simulink model "WarehouseFleetSim"  (R2024b)
settings: Solver=ode4  StartTime=0.0  StopTime=inf  FixedStep=0.02  RelTol=1e-3
StopFcn:
  | try, fleetVisionStep('close'); catch, end; try, phase3('stopped'); catch, end
model workspace (MAT data in the model file):
  HomePose1 = [-20 7.3 0]
  HomePose2 = [-20 3.6 0]
  HomePose3 = [-20 11 0]
  HomePose4 = [-24.5 3.6 0]
  HomePose5 = [-24.5 7.3 0]
  HomePose6 = [-24.5 11 0]
  Zero = 0
  gen3 : robotics.RigidBodyTree (value not decoded)
  qStow = [0; 0; 0.261799387799; 3.14159265359; -2.26892802759; 0; 0.959931088597; 1.57079632679]
undefined symbols (not defined in the file or in its folder): Actor, setupFleetScene, Sim3dSensor, World
libraries: sim3dlib x128, sim3dcameralib x7, robotmobilelib x6, robotsim3dlib x6
(part 2 of 4)

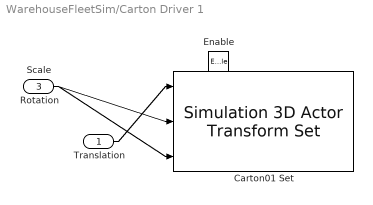
== system WarehouseFleetSim/Carton Driver 1 ==
  Translation : Inport
  Rotation : Inport  Port=2
  Scale : Inport  Port=3
  Enable : EnablePort
  Carton01 Set : sim3dlib/Simulation 3D Actor Transform Set  Priority=1  ActorTag=Carton01  NumberOfParts=1  CustNumOfParts=3  Translation=[0 0 0]  Rotation=[0 0 0]  Scale=[1 1 1]  Ts=-1  aMode=aMode
  wires:
  Translation/1 -> Carton01 Set/1
  Rotation/1 -> Carton01 Set/2
  Scale/1 -> Carton01 Set/3

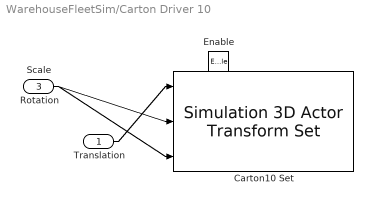
== system WarehouseFleetSim/Carton Driver 10 ==
  Translation : Inport
  Rotation : Inport  Port=2
  Scale : Inport  Port=3
  Enable : EnablePort
  Carton10 Set : sim3dlib/Simulation 3D Actor Transform Set  Priority=1  ActorTag=Carton10  NumberOfParts=1  CustNumOfParts=3  Translation=[0 0 0]  Rotation=[0 0 0]  Scale=[1 1 1]  Ts=-1  aMode=aMode
  wires:
  Translation/1 -> Carton10 Set/1
  Rotation/1 -> Carton10 Set/2
  Scale/1 -> Carton10 Set/3

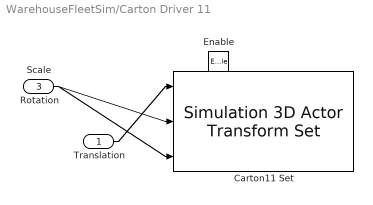
== system WarehouseFleetSim/Carton Driver 11 ==
  Translation : Inport
  Rotation : Inport  Port=2
  Scale : Inport  Port=3
  Enable : EnablePort
  Carton11 Set : sim3dlib/Simulation 3D Actor Transform Set  Priority=1  ActorTag=Carton11  NumberOfParts=1  CustNumOfParts=3  Translation=[0 0 0]  Rotation=[0 0 0]  Scale=[1 1 1]  Ts=-1  aMode=aMode
  wires:
  Translation/1 -> Carton11 Set/1
  Rotation/1 -> Carton11 Set/2
  Scale/1 -> Carton11 Set/3

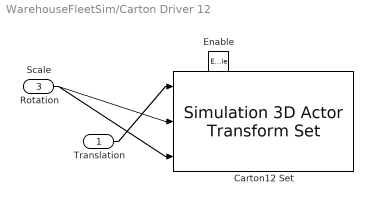
== system WarehouseFleetSim/Carton Driver 12 ==
  Translation : Inport
  Rotation : Inport  Port=2
  Scale : Inport  Port=3
  Enable : EnablePort
  Carton12 Set : sim3dlib/Simulation 3D Actor Transform Set  Priority=1  ActorTag=Carton12  NumberOfParts=1  CustNumOfParts=3  Translation=[0 0 0]  Rotation=[0 0 0]  Scale=[1 1 1]  Ts=-1  aMode=aMode
  wires:
  Translation/1 -> Carton12 Set/1
  Rotation/1 -> Carton12 Set/2
  Scale/1 -> Carton12 Set/3

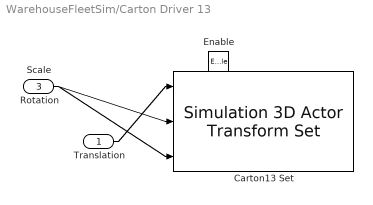
== system WarehouseFleetSim/Carton Driver 13 ==
  Translation : Inport
  Rotation : Inport  Port=2
  Scale : Inport  Port=3
  Enable : EnablePort
  Carton13 Set : sim3dlib/Simulation 3D Actor Transform Set  Priority=1  ActorTag=Carton13  NumberOfParts=1  CustNumOfParts=3  Translation=[0 0 0]  Rotation=[0 0 0]  Scale=[1 1 1]  Ts=-1  aMode=aMode
  wires:
  Translation/1 -> Carton13 Set/1
  Rotation/1 -> Carton13 Set/2
  Scale/1 -> Carton13 Set/3

== system WarehouseFleetSim/Carton Driver 14 ==
  Translation : Inport
  Rotation : Inport  Port=2
  Scale : Inport  Port=3
  Enable : EnablePort
  Carton14 Set : sim3dlib/Simulation 3D Actor Transform Set  Priority=1  ActorTag=Carton14  NumberOfParts=1  CustNumOfParts=3  Translation=[0 0 0]  Rotation=[0 0 0]  Scale=[1 1 1]  Ts=-1  aMode=aMode
  wires:
  Translation/1 -> Carton14 Set/1
  Rotation/1 -> Carton14 Set/2
  Scale/1 -> Carton14 Set/3

== system WarehouseFleetSim/Carton Driver 15 ==
  Translation : Inport
  Rotation : Inport  Port=2
  Scale : Inport  Port=3
  Enable : EnablePort
  Carton15 Set : sim3dlib/Simulation 3D Actor Transform Set  Priority=1  ActorTag=Carton15  NumberOfParts=1  CustNumOfParts=3  Translation=[0 0 0]  Rotation=[0 0 0]  Scale=[1 1 1]  Ts=-1  aMode=aMode
  wires:
  Translation/1 -> Carton15 Set/1
  Rotation/1 -> Carton15 Set/2
  Scale/1 -> Carton15 Set/3

== system WarehouseFleetSim/Carton Driver 16 ==
  Translation : Inport
  Rotation : Inport  Port=2
  Scale : Inport  Port=3
  Enable : EnablePort
  Carton16 Set : sim3dlib/Simulation 3D Actor Transform Set  Priority=1  ActorTag=Carton16  NumberOfParts=1  CustNumOfParts=3  Translation=[0 0 0]  Rotation=[0 0 0]  Scale=[1 1 1]  Ts=-1  aMode=aMode
  wires:
  Translation/1 -> Carton16 Set/1
  Rotation/1 -> Carton16 Set/2
  Scale/1 -> Carton16 Set/3

== system WarehouseFleetSim/Carton Driver 17 ==
  Translation : Inport
  Rotation : Inport  Port=2
  Scale : Inport  Port=3
  Enable : EnablePort
  Carton17 Set : sim3dlib/Simulation 3D Actor Transform Set  Priority=1  ActorTag=Carton17  NumberOfParts=1  CustNumOfParts=3  Translation=[0 0 0]  Rotation=[0 0 0]  Scale=[1 1 1]  Ts=-1  aMode=aMode
  wires:
  Translation/1 -> Carton17 Set/1
  Rotation/1 -> Carton17 Set/2
  Scale/1 -> Carton17 Set/3

== system WarehouseFleetSim/Carton Driver 18 ==
  Translation : Inport
  Rotation : Inport  Port=2
  Scale : Inport  Port=3
  Enable : EnablePort
  Carton18 Set : sim3dlib/Simulation 3D Actor Transform Set  Priority=1  ActorTag=Carton18  NumberOfParts=1  CustNumOfParts=3  Translation=[0 0 0]  Rotation=[0 0 0]  Scale=[1 1 1]  Ts=-1  aMode=aMode
  wires:
  Translation/1 -> Carton18 Set/1
  Rotation/1 -> Carton18 Set/2
  Scale/1 -> Carton18 Set/3

== system WarehouseFleetSim/Carton Driver 19 ==
  Translation : Inport
  Rotation : Inport  Port=2
  Scale : Inport  Port=3
  Enable : EnablePort
  Carton19 Set : sim3dlib/Simulation 3D Actor Transform Set  Priority=1  ActorTag=Carton19  NumberOfParts=1  CustNumOfParts=3  Translation=[0 0 0]  Rotation=[0 0 0]  Scale=[1 1 1]  Ts=-1  aMode=aMode
  wires:
  Translation/1 -> Carton19 Set/1
  Rotation/1 -> Carton19 Set/2
  Scale/1 -> Carton19 Set/3

== system WarehouseFleetSim/Carton Driver 2 ==
  Translation : Inport
  Rotation : Inport  Port=2
  Scale : Inport  Port=3
  Enable : EnablePort
  Carton02 Set : sim3dlib/Simulation 3D Actor Transform Set  Priority=1  ActorTag=Carton02  NumberOfParts=1  CustNumOfParts=3  Translation=[0 0 0]  Rotation=[0 0 0]  Scale=[1 1 1]  Ts=-1  aMode=aMode
  wires:
  Translation/1 -> Carton02 Set/1
  Rotation/1 -> Carton02 Set/2
  Scale/1 -> Carton02 Set/3

== system WarehouseFleetSim/Carton Driver 20 ==
  Translation : Inport
  Rotation : Inport  Port=2
  Scale : Inport  Port=3
  Enable : EnablePort
  Carton20 Set : sim3dlib/Simulation 3D Actor Transform Set  Priority=1  ActorTag=Carton20  NumberOfParts=1  CustNumOfParts=3  Translation=[0 0 0]  Rotation=[0 0 0]  Scale=[1 1 1]  Ts=-1  aMode=aMode
  wires:
  Translation/1 -> Carton20 Set/1
  Rotation/1 -> Carton20 Set/2
  Scale/1 -> Carton20 Set/3

== system WarehouseFleetSim/Carton Driver 21 ==
  Translation : Inport
  Rotation : Inport  Port=2
  Scale : Inport  Port=3
  Enable : EnablePort
  Carton21 Set : sim3dlib/Simulation 3D Actor Transform Set  Priority=1  ActorTag=Carton21  NumberOfParts=1  CustNumOfParts=3  Translation=[0 0 0]  Rotation=[0 0 0]  Scale=[1 1 1]  Ts=-1  aMode=aMode
  wires:
  Translation/1 -> Carton21 Set/1
  Rotation/1 -> Carton21 Set/2
  Scale/1 -> Carton21 Set/3

== system WarehouseFleetSim/Carton Driver 22 ==
  Translation : Inport
  Rotation : Inport  Port=2
  Scale : Inport  Port=3
  Enable : EnablePort
  Carton22 Set : sim3dlib/Simulation 3D Actor Transform Set  Priority=1  ActorTag=Carton22  NumberOfParts=1  CustNumOfParts=3  Translation=[0 0 0]  Rotation=[0 0 0]  Scale=[1 1 1]  Ts=-1  aMode=aMode
  wires:
  Translation/1 -> Carton22 Set/1
  Rotation/1 -> Carton22 Set/2
  Scale/1 -> Carton22 Set/3

== system WarehouseFleetSim/Carton Driver 23 ==
  Translation : Inport
  Rotation : Inport  Port=2
  Scale : Inport  Port=3
  Enable : EnablePort
  Carton23 Set : sim3dlib/Simulation 3D Actor Transform Set  Priority=1  ActorTag=Carton23  NumberOfParts=1  CustNumOfParts=3  Translation=[0 0 0]  Rotation=[0 0 0]  Scale=[1 1 1]  Ts=-1  aMode=aMode
  wires:
  Translation/1 -> Carton23 Set/1
  Rotation/1 -> Carton23 Set/2
  Scale/1 -> Carton23 Set/3

== system WarehouseFleetSim/Carton Driver 24 ==
  Translation : Inport
  Rotation : Inport  Port=2
  Scale : Inport  Port=3
  Enable : EnablePort
  Carton24 Set : sim3dlib/Simulation 3D Actor Transform Set  Priority=1  ActorTag=Carton24  NumberOfParts=1  CustNumOfParts=3  Translation=[0 0 0]  Rotation=[0 0 0]  Scale=[1 1 1]  Ts=-1  aMode=aMode
  wires:
  Translation/1 -> Carton24 Set/1
  Rotation/1 -> Carton24 Set/2
  Scale/1 -> Carton24 Set/3

== system WarehouseFleetSim/Carton Driver 25 ==
  Translation : Inport
  Rotation : Inport  Port=2
  Scale : Inport  Port=3
  Enable : EnablePort
  Carton25 Set : sim3dlib/Simulation 3D Actor Transform Set  Priority=1  ActorTag=Carton25  NumberOfParts=1  CustNumOfParts=3  Translation=[0 0 0]  Rotation=[0 0 0]  Scale=[1 1 1]  Ts=-1  aMode=aMode
  wires:
  Translation/1 -> Carton25 Set/1
  Rotation/1 -> Carton25 Set/2
  Scale/1 -> Carton25 Set/3

== system WarehouseFleetSim/Carton Driver 26 ==
  Translation : Inport
  Rotation : Inport  Port=2
  Scale : Inport  Port=3
  Enable : EnablePort
  Carton26 Set : sim3dlib/Simulation 3D Actor Transform Set  Priority=1  ActorTag=Carton26  NumberOfParts=1  CustNumOfParts=3  Translation=[0 0 0]  Rotation=[0 0 0]  Scale=[1 1 1]  Ts=-1  aMode=aMode
  wires:
  Translation/1 -> Carton26 Set/1
  Rotation/1 -> Carton26 Set/2
  Scale/1 -> Carton26 Set/3

== system WarehouseFleetSim/Carton Driver 27 ==
  Translation : Inport
  Rotation : Inport  Port=2
  Scale : Inport  Port=3
  Enable : EnablePort
  Carton27 Set : sim3dlib/Simulation 3D Actor Transform Set  Priority=1  ActorTag=Carton27  NumberOfParts=1  CustNumOfParts=3  Translation=[0 0 0]  Rotation=[0 0 0]  Scale=[1 1 1]  Ts=-1  aMode=aMode
  wires:
  Translation/1 -> Carton27 Set/1
  Rotation/1 -> Carton27 Set/2
  Scale/1 -> Carton27 Set/3

== system WarehouseFleetSim/Carton Driver 28 ==
  Translation : Inport
  Rotation : Inport  Port=2
  Scale : Inport  Port=3
  Enable : EnablePort
  Carton28 Set : sim3dlib/Simulation 3D Actor Transform Set  Priority=1  ActorTag=Carton28  NumberOfParts=1  CustNumOfParts=3  Translation=[0 0 0]  Rotation=[0 0 0]  Scale=[1 1 1]  Ts=-1  aMode=aMode
  wires:
  Translation/1 -> Carton28 Set/1
  Rotation/1 -> Carton28 Set/2
  Scale/1 -> Carton28 Set/3

== system WarehouseFleetSim/Carton Driver 29 ==
  Translation : Inport
  Rotation : Inport  Port=2
  Scale : Inport  Port=3
  Enable : EnablePort
  Carton29 Set : sim3dlib/Simulation 3D Actor Transform Set  Priority=1  ActorTag=Carton29  NumberOfParts=1  CustNumOfParts=3  Translation=[0 0 0]  Rotation=[0 0 0]  Scale=[1 1 1]  Ts=-1  aMode=aMode
  wires:
  Translation/1 -> Carton29 Set/1
  Rotation/1 -> Carton29 Set/2
  Scale/1 -> Carton29 Set/3

== system WarehouseFleetSim/Carton Driver 3 ==
  Translation : Inport
  Rotation : Inport  Port=2
  Scale : Inport  Port=3
  Enable : EnablePort
  Carton03 Set : sim3dlib/Simulation 3D Actor Transform Set  Priority=1  ActorTag=Carton03  NumberOfParts=1  CustNumOfParts=3  Translation=[0 0 0]  Rotation=[0 0 0]  Scale=[1 1 1]  Ts=-1  aMode=aMode
  wires:
  Translation/1 -> Carton03 Set/1
  Rotation/1 -> Carton03 Set/2
  Scale/1 -> Carton03 Set/3

== system WarehouseFleetSim/Carton Driver 30 ==
  Translation : Inport
  Rotation : Inport  Port=2
  Scale : Inport  Port=3
  Enable : EnablePort
  Carton30 Set : sim3dlib/Simulation 3D Actor Transform Set  Priority=1  ActorTag=Carton30  NumberOfParts=1  CustNumOfParts=3  Translation=[0 0 0]  Rotation=[0 0 0]  Scale=[1 1 1]  Ts=-1  aMode=aMode
  wires:
  Translation/1 -> Carton30 Set/1
  Rotation/1 -> Carton30 Set/2
  Scale/1 -> Carton30 Set/3

== system WarehouseFleetSim/Carton Driver 31 ==
  Translation : Inport
  Rotation : Inport  Port=2
  Scale : Inport  Port=3
  Enable : EnablePort
  Carton31 Set : sim3dlib/Simulation 3D Actor Transform Set  Priority=1  ActorTag=Carton31  NumberOfParts=1  CustNumOfParts=3  Translation=[0 0 0]  Rotation=[0 0 0]  Scale=[1 1 1]  Ts=-1  aMode=aMode
  wires:
  Translation/1 -> Carton31 Set/1
  Rotation/1 -> Carton31 Set/2
  Scale/1 -> Carton31 Set/3

== system WarehouseFleetSim/Carton Driver 32 ==
  Translation : Inport
  Rotation : Inport  Port=2
  Scale : Inport  Port=3
  Enable : EnablePort
  Carton32 Set : sim3dlib/Simulation 3D Actor Transform Set  Priority=1  ActorTag=Carton32  NumberOfParts=1  CustNumOfParts=3  Translation=[0 0 0]  Rotation=[0 0 0]  Scale=[1 1 1]  Ts=-1  aMode=aMode
  wires:
  Translation/1 -> Carton32 Set/1
  Rotation/1 -> Carton32 Set/2
  Scale/1 -> Carton32 Set/3

== system WarehouseFleetSim/Carton Driver 33 ==
  Translation : Inport
  Rotation : Inport  Port=2
  Scale : Inport  Port=3
  Enable : EnablePort
  Carton33 Set : sim3dlib/Simulation 3D Actor Transform Set  Priority=1  ActorTag=Carton33  NumberOfParts=1  CustNumOfParts=3  Translation=[0 0 0]  Rotation=[0 0 0]  Scale=[1 1 1]  Ts=-1  aMode=aMode
  wires:
  Translation/1 -> Carton33 Set/1
  Rotation/1 -> Carton33 Set/2
  Scale/1 -> Carton33 Set/3

== system WarehouseFleetSim/Carton Driver 34 ==
  Translation : Inport
  Rotation : Inport  Port=2
  Scale : Inport  Port=3
  Enable : EnablePort
  Carton34 Set : sim3dlib/Simulation 3D Actor Transform Set  Priority=1  ActorTag=Carton34  NumberOfParts=1  CustNumOfParts=3  Translation=[0 0 0]  Rotation=[0 0 0]  Scale=[1 1 1]  Ts=-1  aMode=aMode
  wires:
  Translation/1 -> Carton34 Set/1
  Rotation/1 -> Carton34 Set/2
  Scale/1 -> Carton34 Set/3

== system WarehouseFleetSim/Carton Driver 35 ==
  Translation : Inport
  Rotation : Inport  Port=2
  Scale : Inport  Port=3
  Enable : EnablePort
  Carton35 Set : sim3dlib/Simulation 3D Actor Transform Set  Priority=1  ActorTag=Carton35  NumberOfParts=1  CustNumOfParts=3  Translation=[0 0 0]  Rotation=[0 0 0]  Scale=[1 1 1]  Ts=-1  aMode=aMode
  wires:
  Translation/1 -> Carton35 Set/1
  Rotation/1 -> Carton35 Set/2
  Scale/1 -> Carton35 Set/3

== system WarehouseFleetSim/Carton Driver 36 ==
  Translation : Inport
  Rotation : Inport  Port=2
  Scale : Inport  Port=3
  Enable : EnablePort
  Carton36 Set : sim3dlib/Simulation 3D Actor Transform Set  Priority=1  ActorTag=Carton36  NumberOfParts=1  CustNumOfParts=3  Translation=[0 0 0]  Rotation=[0 0 0]  Scale=[1 1 1]  Ts=-1  aMode=aMode
  wires:
  Translation/1 -> Carton36 Set/1
  Rotation/1 -> Carton36 Set/2
  Scale/1 -> Carton36 Set/3

== system WarehouseFleetSim/Carton Driver 37 ==
  Translation : Inport
  Rotation : Inport  Port=2
  Scale : Inport  Port=3
  Enable : EnablePort
  Carton37 Set : sim3dlib/Simulation 3D Actor Transform Set  Priority=1  ActorTag=Carton37  NumberOfParts=1  CustNumOfParts=3  Translation=[0 0 0]  Rotation=[0 0 0]  Scale=[1 1 1]  Ts=-1  aMode=aMode
  wires:
  Translation/1 -> Carton37 Set/1
  Rotation/1 -> Carton37 Set/2
  Scale/1 -> Carton37 Set/3

== system WarehouseFleetSim/Carton Driver 38 ==
  Translation : Inport
  Rotation : Inport  Port=2
  Scale : Inport  Port=3
  Enable : EnablePort
  Carton38 Set : sim3dlib/Simulation 3D Actor Transform Set  Priority=1  ActorTag=Carton38  NumberOfParts=1  CustNumOfParts=3  Translation=[0 0 0]  Rotation=[0 0 0]  Scale=[1 1 1]  Ts=-1  aMode=aMode
  wires:
  Translation/1 -> Carton38 Set/1
  Rotation/1 -> Carton38 Set/2
  Scale/1 -> Carton38 Set/3

== system WarehouseFleetSim/Carton Driver 39 ==
  Translation : Inport
  Rotation : Inport  Port=2
  Scale : Inport  Port=3
  Enable : EnablePort
  Carton39 Set : sim3dlib/Simulation 3D Actor Transform Set  Priority=1  ActorTag=Carton39  NumberOfParts=1  CustNumOfParts=3  Translation=[0 0 0]  Rotation=[0 0 0]  Scale=[1 1 1]  Ts=-1  aMode=aMode
  wires:
  Translation/1 -> Carton39 Set/1
  Rotation/1 -> Carton39 Set/2
  Scale/1 -> Carton39 Set/3

== system WarehouseFleetSim/Carton Driver 4 ==
  Translation : Inport
  Rotation : Inport  Port=2
  Scale : Inport  Port=3
  Enable : EnablePort
  Carton04 Set : sim3dlib/Simulation 3D Actor Transform Set  Priority=1  ActorTag=Carton04  NumberOfParts=1  CustNumOfParts=3  Translation=[0 0 0]  Rotation=[0 0 0]  Scale=[1 1 1]  Ts=-1  aMode=aMode
  wires:
  Translation/1 -> Carton04 Set/1
  Rotation/1 -> Carton04 Set/2
  Scale/1 -> Carton04 Set/3

== system WarehouseFleetSim/Carton Driver 40 ==
  Translation : Inport
  Rotation : Inport  Port=2
  Scale : Inport  Port=3
  Enable : EnablePort
  Carton40 Set : sim3dlib/Simulation 3D Actor Transform Set  Priority=1  ActorTag=Carton40  NumberOfParts=1  CustNumOfParts=3  Translation=[0 0 0]  Rotation=[0 0 0]  Scale=[1 1 1]  Ts=-1  aMode=aMode
  wires:
  Translation/1 -> Carton40 Set/1
  Rotation/1 -> Carton40 Set/2
  Scale/1 -> Carton40 Set/3

== system WarehouseFleetSim/Carton Driver 41 ==
  Translation : Inport
  Rotation : Inport  Port=2
  Scale : Inport  Port=3
  Enable : EnablePort
  Carton41 Set : sim3dlib/Simulation 3D Actor Transform Set  Priority=1  ActorTag=Carton41  NumberOfParts=1  CustNumOfParts=3  Translation=[0 0 0]  Rotation=[0 0 0]  Scale=[1 1 1]  Ts=-1  aMode=aMode
  wires:
  Translation/1 -> Carton41 Set/1
  Rotation/1 -> Carton41 Set/2
  Scale/1 -> Carton41 Set/3

== system WarehouseFleetSim/Carton Driver 42 ==
  Translation : Inport
  Rotation : Inport  Port=2
  Scale : Inport  Port=3
  Enable : EnablePort
  Carton42 Set : sim3dlib/Simulation 3D Actor Transform Set  Priority=1  ActorTag=Carton42  NumberOfParts=1  CustNumOfParts=3  Translation=[0 0 0]  Rotation=[0 0 0]  Scale=[1 1 1]  Ts=-1  aMode=aMode
  wires:
  Translation/1 -> Carton42 Set/1
  Rotation/1 -> Carton42 Set/2
  Scale/1 -> Carton42 Set/3

== system WarehouseFleetSim/Carton Driver 43 ==
  Translation : Inport
  Rotation : Inport  Port=2
  Scale : Inport  Port=3
  Enable : EnablePort
  Carton43 Set : sim3dlib/Simulation 3D Actor Transform Set  Priority=1  ActorTag=Carton43  NumberOfParts=1  CustNumOfParts=3  Translation=[0 0 0]  Rotation=[0 0 0]  Scale=[1 1 1]  Ts=-1  aMode=aMode
  wires:
  Translation/1 -> Carton43 Set/1
  Rotation/1 -> Carton43 Set/2
  Scale/1 -> Carton43 Set/3

== system WarehouseFleetSim/Carton Driver 44 ==
  Translation : Inport
  Rotation : Inport  Port=2
  Scale : Inport  Port=3
  Enable : EnablePort
  Carton44 Set : sim3dlib/Simulation 3D Actor Transform Set  Priority=1  ActorTag=Carton44  NumberOfParts=1  CustNumOfParts=3  Translation=[0 0 0]  Rotation=[0 0 0]  Scale=[1 1 1]  Ts=-1  aMode=aMode
  wires:
  Translation/1 -> Carton44 Set/1
  Rotation/1 -> Carton44 Set/2
  Scale/1 -> Carton44 Set/3

== system WarehouseFleetSim/Carton Driver 45 ==
  Translation : Inport
  Rotation : Inport  Port=2
  Scale : Inport  Port=3
  Enable : EnablePort
  Carton45 Set : sim3dlib/Simulation 3D Actor Transform Set  Priority=1  ActorTag=Carton45  NumberOfParts=1  CustNumOfParts=3  Translation=[0 0 0]  Rotation=[0 0 0]  Scale=[1 1 1]  Ts=-1  aMode=aMode
  wires:
  Translation/1 -> Carton45 Set/1
  Rotation/1 -> Carton45 Set/2
  Scale/1 -> Carton45 Set/3

== system WarehouseFleetSim/Carton Driver 46 ==
  Translation : Inport
  Rotation : Inport  Port=2
  Scale : Inport  Port=3
  Enable : EnablePort
  Carton46 Set : sim3dlib/Simulation 3D Actor Transform Set  Priority=1  ActorTag=Carton46  NumberOfParts=1  CustNumOfParts=3  Translation=[0 0 0]  Rotation=[0 0 0]  Scale=[1 1 1]  Ts=-1  aMode=aMode
  wires:
  Translation/1 -> Carton46 Set/1
  Rotation/1 -> Carton46 Set/2
  Scale/1 -> Carton46 Set/3

== system WarehouseFleetSim/Carton Driver 47 ==
  Translation : Inport
  Rotation : Inport  Port=2
  Scale : Inport  Port=3
  Enable : EnablePort
  Carton47 Set : sim3dlib/Simulation 3D Actor Transform Set  Priority=1  ActorTag=Carton47  NumberOfParts=1  CustNumOfParts=3  Translation=[0 0 0]  Rotation=[0 0 0]  Scale=[1 1 1]  Ts=-1  aMode=aMode
  wires:
  Translation/1 -> Carton47 Set/1
  Rotation/1 -> Carton47 Set/2
  Scale/1 -> Carton47 Set/3

== system WarehouseFleetSim/Carton Driver 48 ==
  Translation : Inport
  Rotation : Inport  Port=2
  Scale : Inport  Port=3
  Enable : EnablePort
  Carton48 Set : sim3dlib/Simulation 3D Actor Transform Set  Priority=1  ActorTag=Carton48  NumberOfParts=1  CustNumOfParts=3  Translation=[0 0 0]  Rotation=[0 0 0]  Scale=[1 1 1]  Ts=-1  aMode=aMode
  wires:
  Translation/1 -> Carton48 Set/1
  Rotation/1 -> Carton48 Set/2
  Scale/1 -> Carton48 Set/3

== system WarehouseFleetSim/Carton Driver 49 ==
  Translation : Inport
  Rotation : Inport  Port=2
  Scale : Inport  Port=3
  Enable : EnablePort
  Carton49 Set : sim3dlib/Simulation 3D Actor Transform Set  Priority=1  ActorTag=Carton49  NumberOfParts=1  CustNumOfParts=3  Translation=[0 0 0]  Rotation=[0 0 0]  Scale=[1 1 1]  Ts=-1  aMode=aMode
  wires:
  Translation/1 -> Carton49 Set/1
  Rotation/1 -> Carton49 Set/2
  Scale/1 -> Carton49 Set/3

== system WarehouseFleetSim/Carton Driver 5 ==
  Translation : Inport
  Rotation : Inport  Port=2
  Scale : Inport  Port=3
  Enable : EnablePort
  Carton05 Set : sim3dlib/Simulation 3D Actor Transform Set  Priority=1  ActorTag=Carton05  NumberOfParts=1  CustNumOfParts=3  Translation=[0 0 0]  Rotation=[0 0 0]  Scale=[1 1 1]  Ts=-1  aMode=aMode
  wires:
  Translation/1 -> Carton05 Set/1
  Rotation/1 -> Carton05 Set/2
  Scale/1 -> Carton05 Set/3

== system WarehouseFleetSim/Carton Driver 50 ==
  Translation : Inport
  Rotation : Inport  Port=2
  Scale : Inport  Port=3
  Enable : EnablePort
  Carton50 Set : sim3dlib/Simulation 3D Actor Transform Set  Priority=1  ActorTag=Carton50  NumberOfParts=1  CustNumOfParts=3  Translation=[0 0 0]  Rotation=[0 0 0]  Scale=[1 1 1]  Ts=-1  aMode=aMode
  wires:
  Translation/1 -> Carton50 Set/1
  Rotation/1 -> Carton50 Set/2
  Scale/1 -> Carton50 Set/3

== system WarehouseFleetSim/Carton Driver 51 ==
  Translation : Inport
  Rotation : Inport  Port=2
  Scale : Inport  Port=3
  Enable : EnablePort
  Carton51 Set : sim3dlib/Simulation 3D Actor Transform Set  Priority=1  ActorTag=Carton51  NumberOfParts=1  CustNumOfParts=3  Translation=[0 0 0]  Rotation=[0 0 0]  Scale=[1 1 1]  Ts=-1  aMode=aMode
  wires:
  Translation/1 -> Carton51 Set/1
  Rotation/1 -> Carton51 Set/2
  Scale/1 -> Carton51 Set/3

== system WarehouseFleetSim/Carton Driver 52 ==
  Translation : Inport
  Rotation : Inport  Port=2
  Scale : Inport  Port=3
  Enable : EnablePort
  Carton52 Set : sim3dlib/Simulation 3D Actor Transform Set  Priority=1  ActorTag=Carton52  NumberOfParts=1  CustNumOfParts=3  Translation=[0 0 0]  Rotation=[0 0 0]  Scale=[1 1 1]  Ts=-1  aMode=aMode
  wires:
  Translation/1 -> Carton52 Set/1
  Rotation/1 -> Carton52 Set/2
  Scale/1 -> Carton52 Set/3

== system WarehouseFleetSim/Carton Driver 53 ==
  Translation : Inport
  Rotation : Inport  Port=2
  Scale : Inport  Port=3
  Enable : EnablePort
  Carton53 Set : sim3dlib/Simulation 3D Actor Transform Set  Priority=1  ActorTag=Carton53  NumberOfParts=1  CustNumOfParts=3  Translation=[0 0 0]  Rotation=[0 0 0]  Scale=[1 1 1]  Ts=-1  aMode=aMode
  wires:
  Translation/1 -> Carton53 Set/1
  Rotation/1 -> Carton53 Set/2
  Scale/1 -> Carton53 Set/3

== system WarehouseFleetSim/Carton Driver 54 ==
  Translation : Inport
  Rotation : Inport  Port=2
  Scale : Inport  Port=3
  Enable : EnablePort
  Carton54 Set : sim3dlib/Simulation 3D Actor Transform Set  Priority=1  ActorTag=Carton54  NumberOfParts=1  CustNumOfParts=3  Translation=[0 0 0]  Rotation=[0 0 0]  Scale=[1 1 1]  Ts=-1  aMode=aMode
  wires:
  Translation/1 -> Carton54 Set/1
  Rotation/1 -> Carton54 Set/2
  Scale/1 -> Carton54 Set/3

== system WarehouseFleetSim/Carton Driver 6 ==
  Translation : Inport
  Rotation : Inport  Port=2
  Scale : Inport  Port=3
  Enable : EnablePort
  Carton06 Set : sim3dlib/Simulation 3D Actor Transform Set  Priority=1  ActorTag=Carton06  NumberOfParts=1  CustNumOfParts=3  Translation=[0 0 0]  Rotation=[0 0 0]  Scale=[1 1 1]  Ts=-1  aMode=aMode
  wires:
  Translation/1 -> Carton06 Set/1
  Rotation/1 -> Carton06 Set/2
  Scale/1 -> Carton06 Set/3

== system WarehouseFleetSim/Carton Driver 7 ==
  Translation : Inport
  Rotation : Inport  Port=2
  Scale : Inport  Port=3
  Enable : EnablePort
  Carton07 Set : sim3dlib/Simulation 3D Actor Transform Set  Priority=1  ActorTag=Carton07  NumberOfParts=1  CustNumOfParts=3  Translation=[0 0 0]  Rotation=[0 0 0]  Scale=[1 1 1]  Ts=-1  aMode=aMode
  wires:
  Translation/1 -> Carton07 Set/1
  Rotation/1 -> Carton07 Set/2
  Scale/1 -> Carton07 Set/3

== system WarehouseFleetSim/Carton Driver 8 ==
  Translation : Inport
  Rotation : Inport  Port=2
  Scale : Inport  Port=3
  Enable : EnablePort
  Carton08 Set : sim3dlib/Simulation 3D Actor Transform Set  Priority=1  ActorTag=Carton08  NumberOfParts=1  CustNumOfParts=3  Translation=[0 0 0]  Rotation=[0 0 0]  Scale=[1 1 1]  Ts=-1  aMode=aMode
  wires:
  Translation/1 -> Carton08 Set/1
  Rotation/1 -> Carton08 Set/2
  Scale/1 -> Carton08 Set/3

== system WarehouseFleetSim/Carton Driver 9 ==
  Translation : Inport
  Rotation : Inport  Port=2
  Scale : Inport  Port=3
  Enable : EnablePort
  Carton09 Set : sim3dlib/Simulation 3D Actor Transform Set  Priority=1  ActorTag=Carton09  NumberOfParts=1  CustNumOfParts=3  Translation=[0 0 0]  Rotation=[0 0 0]  Scale=[1 1 1]  Ts=-1  aMode=aMode
  wires:
  Translation/1 -> Carton09 Set/1
  Rotation/1 -> Carton09 Set/2
  Scale/1 -> Carton09 Set/3

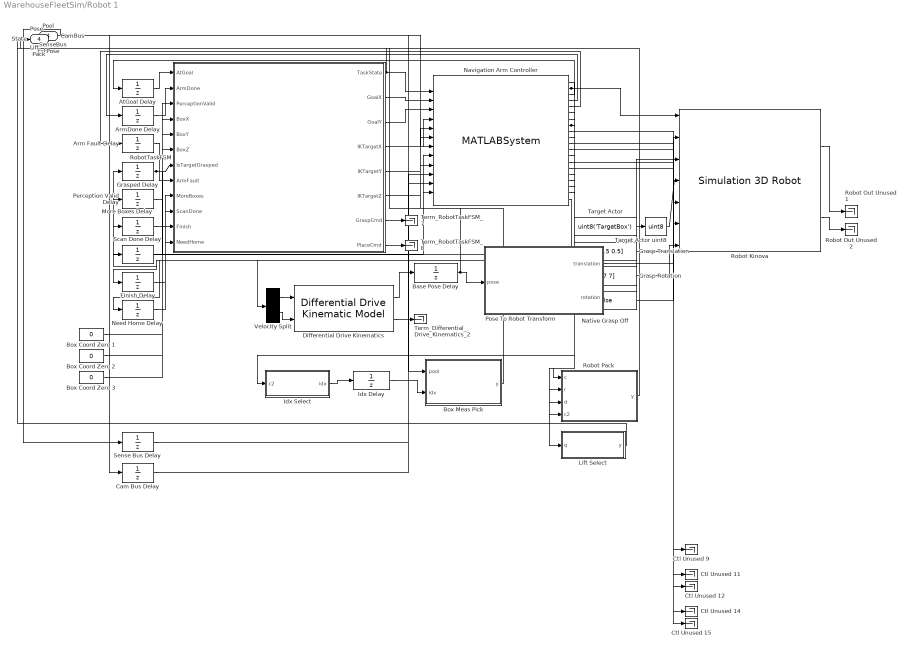
== system WarehouseFleetSim/Robot 1 ==
  Pool : Inport
  EstPose : Inport  Port=2
  SenseBus : Inport  Port=3
  CamBus : Inport  Port=4
  Arm Fault Delay : UnitDelay  InitialCondition=false  SampleTime=0.02  HasFrameUpgradeWarning=on
  ArmDone Delay : UnitDelay  InitialCondition=false  SampleTime=0.02  HasFrameUpgradeWarning=on
  AtGoal Delay : UnitDelay  InitialCondition=false  SampleTime=0.02  HasFrameUpgradeWarning=on
  Base Pose Delay : UnitDelay  InitialCondition=HomePose1  SampleTime=0.02  HasFrameUpgradeWarning=on
  Box Coord Zero 1 : Constant  Value=0  OutDataTypeStr=double
  Box Coord Zero 2 : Constant  Value=0  OutDataTypeStr=double
  Box Coord Zero 3 : Constant  Value=0  OutDataTypeStr=double
  Box Meas Pick : MATLAB Function  TreatAsAtomicUnit=on
  Cam Bus Delay : UnitDelay  InitialCondition=zeros(1,8)  SampleTime=0.02  HasFrameUpgradeWarning=on
  Ctl Unused {9,11..12,14..15} (5 alike) : Terminator
  Differential Drive Kinematics : robotmobilelib/Differential Drive Kinematic Model  VehicleInputs=Vehicle Speed & Heading Angular Velocity  WheelRadius=0.05  WheelSpeedRange=[-inf inf]  TrackWidth=0.2  InitialState=HomePose1  SimulateUsing=Interpreted execution
  Finish Delay : UnitDelay  InitialCondition=false  SampleTime=0.02  HasFrameUpgradeWarning=on
  Grasp Rotation : Constant  Value=[7 7 7]
  Grasp Translation : Constant  Value=[0.5 0.5 0.5]
  Grasped Delay : UnitDelay  InitialCondition=false  SampleTime=0.02  HasFrameUpgradeWarning=on
  Idx Delay : UnitDelay  SampleTime=0.02  HasFrameUpgradeWarning=on
  Idx Select : MATLAB Function  TreatAsAtomicUnit=on
  Lift Select : MATLAB Function  TreatAsAtomicUnit=on
  More Boxes Delay : UnitDelay  InitialCondition=false  SampleTime=0.02  HasFrameUpgradeWarning=on
  Native Grasp Off : Constant  Value=false  OutDataTypeStr=boolean
  Navigation Arm Controller : MATLABSystem  System=WarehouseRobotControlSystemV23  SampleTime=0.02  RobotId=1  SimulateUsing=Interpreted execution
      mask Type: WarehouseRobotControlSystemV23
      mask Display:
      | disp('WarehouseRobotControlSystemV23');
      | port_label('input',1,'state');
      | port_label('input',2,'~');
      | port_label('input',3,'~');
      | port_label('input',4,'~');
      | port_label('input',5,'~');
      | port_label('input',6,'~');
      | port_label('input',7,'basePose');
      | port_label('input',8,'isTargetGrasped');
      | port_label('input',9,'boxMeas');
      | port_label('input',10,'senseBus');
      | port_label('input',11,'camBus');
      | port_label('input',12,'truePose');
      | port_label('output',1,'velocity');
      | port_label('output',2,'config');
      | port_label('output',3,'atGoal');
      | port_label('output',4,'armDone');
      | port_label('output',5,'armFault');
      | port_label('output',6,'vacuum');
      | port_label('output',7,'c1');
      | port_label('output',8,'c2');
      | port_label('output',9,'c3');
      | port_label('output',10,'r1');
      | port_label('output',11,'r2');
      | port_label('output',12,'r3');
      | port_label('output',13,'d1');
      | port_label('output',14,'d2');
      | port_label('output',15,'d3');
      | port_label('output',16,'percValid');
      | port_label('output',17,'moreBoxes');
      | port_label('output',18,'scanDone');
      | port_label('output',19,'finish');
      | port_label('output',20,'needHome');
  Need Home Delay : UnitDelay  InitialCondition=false  SampleTime=0.02  HasFrameUpgradeWarning=on
  Perception Valid Delay : UnitDelay  InitialCondition=false  SampleTime=0.02  HasFrameUpgradeWarning=on
  Pose To Robot Transform : MATLAB Function  TreatAsAtomicUnit=on
  Robot Kinova : robotsim3dlib/Simulation 3D Robot  Priority=2  actorInputType=RigidBodyTree Object  RigidBodyTree=gen3  ActorName=Ro1Kinova  existActorChekBox=off  initialTrans=[0 0 0]  initialRot=[0 0 0]  initialConfig=qStow  EndEffector=ToolTip  eeOffsetInpChekBox=off  eeTargetTrans=[-0.04 0 0.245]  eeTargetRot=[0 1.2217 3.1416]  enableRegionGraspChekBox=on  regionGraspInpChekBox=on  eeTargTransDiff=[0.2 0.2 0.2]  eeTargRotDiff=[0 0 0]  inpConfEnbVal=on  inpGraspEnbVal=on  inpTransEnbVal=on  outConfEnbVal=on  outGraspEnbVal=on  outTransEnbVal=off  SampleTime=0.02  ActorType=SimulinkVehicle  ID=C  aMode=6  ActorTag=Ro1Kinova  Mesh=RigidBodyTree
  Robot Out Unused 1 : Terminator
  Robot Out Unused 2 : Terminator
  Robot Pack : MATLAB Function  TreatAsAtomicUnit=on
  RobotTaskFSM : Stateflow chart  TreatAsAtomicUnit=on
  Scan Done Delay : UnitDelay  InitialCondition=false  SampleTime=0.02  HasFrameUpgradeWarning=on
  Sense Bus Delay : UnitDelay  InitialCondition=zeros(1,8)  SampleTime=0.02  HasFrameUpgradeWarning=on
  Target Actor : Constant  Value=uint8('TargetBox')  OutDataTypeStr=uint8
  Target Actor uint8 : DataTypeConversion  OutDataTypeStr=uint8  SaturateOnIntegerOverflow=off  RndMeth=Floor
  Term_Differential_Drive_Kinematics_2 : Terminator
  Term_RobotTaskFSM_7 : Terminator
  Term_RobotTaskFSM_8 : Terminator
  Velocity Split : Demux  Outputs=2
  Pose : Outport
  Pack : Outport  Port=2
  Lift : Outport  Port=3
  State : Outport  Port=4
  wires:
  Navigation Arm Controller/3 -> AtGoal Delay/1
  AtGoal Delay/1 -> RobotTaskFSM/1(AtGoal)
  Navigation Arm Controller/4 -> ArmDone Delay/1
  ArmDone Delay/1 -> RobotTaskFSM/2(ArmDone)
  Navigation Arm Controller/5 -> Arm Fault Delay/1
  Arm Fault Delay/1 -> RobotTaskFSM/8(ArmFault)
  Navigation Arm Controller/6 -> Grasped Delay/1
  Grasped Delay/1 -> RobotTaskFSM/7(IsTargetGrasped), Navigation Arm Controller/8
  Navigation Arm Controller/16 -> Perception Valid Delay/1
  Perception Valid Delay/1 -> RobotTaskFSM/3(PerceptionValid)
  Navigation Arm Controller/17 -> More Boxes Delay/1
  More Boxes Delay/1 -> RobotTaskFSM/9(MoreBoxes)
  Navigation Arm Controller/18 -> Scan Done Delay/1
  Scan Done Delay/1 -> RobotTaskFSM/10(ScanDone)
  Navigation Arm Controller/19 -> Finish Delay/1
  Finish Delay/1 -> RobotTaskFSM/11(Finish)
  Navigation Arm Controller/20 -> Need Home Delay/1
  Need Home Delay/1 -> RobotTaskFSM/12(NeedHome)
  Box Coord Zero 1/1 -> RobotTaskFSM/4(BoxX)
  Box Coord Zero 2/1 -> RobotTaskFSM/5(BoxY)
  Box Coord Zero 3/1 -> RobotTaskFSM/6(BoxZ)
  RobotTaskFSM/1(TaskState) -> Navigation Arm Controller/1, State/1
  RobotTaskFSM/2(GoalX) -> Navigation Arm Controller/2
  RobotTaskFSM/3(GoalY) -> Navigation Arm Controller/3
  RobotTaskFSM/4(IKTargetX) -> Navigation Arm Controller/4
  RobotTaskFSM/5(IKTargetY) -> Navigation Arm Controller/5
  RobotTaskFSM/6(IKTargetZ) -> Navigation Arm Controller/6
  EstPose/1 -> Navigation Arm Controller/7
  SenseBus/1 -> Sense Bus Delay/1
  Sense Bus Delay/1 -> Navigation Arm Controller/10
  CamBus/1 -> Cam Bus Delay/1
  Cam Bus Delay/1 -> Navigation Arm Controller/11
  Base Pose Delay/1 -> Navigation Arm Controller/12, Pose/1, Pose To Robot Transform/1(pose)
  Navigation Arm Controller/8 -> Idx Select/1(c2), Robot Pack/4(c2)
  Idx Select/1(idx) -> Idx Delay/1
  Idx Delay/1 -> Box Meas Pick/2(idx)
  Pool/1 -> Box Meas Pick/1(pool)
  Box Meas Pick/1(y) -> Navigation Arm Controller/9
  Navigation Arm Controller/7 -> Robot Pack/1(c)
  Navigation Arm Controller/10 -> Robot Pack/2(r)
  Navigation Arm Controller/13 -> Robot Pack/3(d)
  Robot Pack/1(y) -> Pack/1
  Navigation Arm Controller/2 -> Lift Select/1(q), Robot Kinova/1
  Lift Select/1(y) -> Lift/1
  Navigation Arm Controller/9 -> Ctl Unused 9/1
  Navigation Arm Controller/11 -> Ctl Unused 11/1
  Navigation Arm Controller/12 -> Ctl Unused 12/1
  Navigation Arm Controller/14 -> Ctl Unused 14/1
  Navigation Arm Controller/15 -> Ctl Unused 15/1
  Navigation Arm Controller/1 -> Velocity Split/1
  Velocity Split/1 -> Differential Drive Kinematics/1
  Velocity Split/2 -> Differential Drive Kinematics/2
  Differential Drive Kinematics/1 -> Base Pose Delay/1
  Target Actor/1 -> Target Actor uint8/1
  Pose To Robot Transform/1(translation) -> Robot Kinova/2
  Pose To Robot Transform/2(rotation) -> Robot Kinova/3
  Target Actor uint8/1 -> Robot Kinova/4
  Native Grasp Off/1 -> Robot Kinova/5
  Grasp Translation/1 -> Robot Kinova/6
  Grasp Rotation/1 -> Robot Kinova/7
  Robot Kinova/1 -> Robot Out Unused 1/1
  Robot Kinova/2 -> Robot Out Unused 2/1
  Differential Drive Kinematics/2 -> Term_Differential_Drive_Kinematics_2/1
  RobotTaskFSM/7(GraspCmd) -> Term_RobotTaskFSM_7/1
  RobotTaskFSM/8(PlaceCmd) -> Term_RobotTaskFSM_8/1

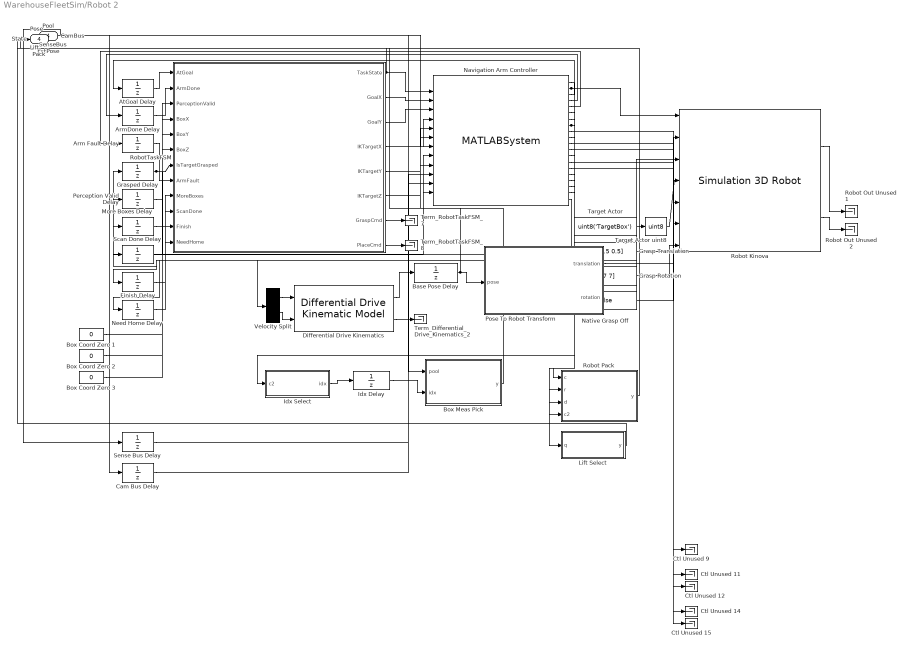
== system WarehouseFleetSim/Robot 2 ==
  Pool : Inport
  EstPose : Inport  Port=2
  SenseBus : Inport  Port=3
  CamBus : Inport  Port=4
  Arm Fault Delay : UnitDelay  InitialCondition=false  SampleTime=0.02  HasFrameUpgradeWarning=on
  ArmDone Delay : UnitDelay  InitialCondition=false  SampleTime=0.02  HasFrameUpgradeWarning=on
  AtGoal Delay : UnitDelay  InitialCondition=false  SampleTime=0.02  HasFrameUpgradeWarning=on
  Base Pose Delay : UnitDelay  InitialCondition=HomePose2  SampleTime=0.02  HasFrameUpgradeWarning=on
  Box Coord Zero 1 : Constant  Value=0  OutDataTypeStr=double
  Box Coord Zero 2 : Constant  Value=0  OutDataTypeStr=double
  Box Coord Zero 3 : Constant  Value=0  OutDataTypeStr=double
  Box Meas Pick : MATLAB Function  TreatAsAtomicUnit=on
  Cam Bus Delay : UnitDelay  InitialCondition=zeros(1,8)  SampleTime=0.02  HasFrameUpgradeWarning=on
  Ctl Unused {9,11..12,14..15} (5 alike) : Terminator
  Differential Drive Kinematics : robotmobilelib/Differential Drive Kinematic Model  VehicleInputs=Vehicle Speed & Heading Angular Velocity  WheelRadius=0.05  WheelSpeedRange=[-inf inf]  TrackWidth=0.2  InitialState=HomePose2  SimulateUsing=Interpreted execution
  Finish Delay : UnitDelay  InitialCondition=false  SampleTime=0.02  HasFrameUpgradeWarning=on
  Grasp Rotation : Constant  Value=[7 7 7]
  Grasp Translation : Constant  Value=[0.5 0.5 0.5]
  Grasped Delay : UnitDelay  InitialCondition=false  SampleTime=0.02  HasFrameUpgradeWarning=on
  Idx Delay : UnitDelay  SampleTime=0.02  HasFrameUpgradeWarning=on
  Idx Select : MATLAB Function  TreatAsAtomicUnit=on
  Lift Select : MATLAB Function  TreatAsAtomicUnit=on
  More Boxes Delay : UnitDelay  InitialCondition=false  SampleTime=0.02  HasFrameUpgradeWarning=on
  Native Grasp Off : Constant  Value=false  OutDataTypeStr=boolean
  Navigation Arm Controller : MATLABSystem  System=WarehouseRobotControlSystemV23  SampleTime=0.02  RobotId=2  SimulateUsing=Interpreted execution
      mask Type: WarehouseRobotControlSystemV23
      mask Display:
      | disp('WarehouseRobotControlSystemV23');
      | port_label('input',1,'state');
      | port_label('input',2,'~');
      | port_label('input',3,'~');
      | port_label('input',4,'~');
      | port_label('input',5,'~');
      | port_label('input',6,'~');
      | port_label('input',7,'basePose');
      | port_label('input',8,'isTargetGrasped');
      | port_label('input',9,'boxMeas');
      | port_label('input',10,'senseBus');
      | port_label('input',11,'camBus');
      | port_label('input',12,'truePose');
      | port_label('output',1,'velocity');
      | port_label('output',2,'config');
      | port_label('output',3,'atGoal');
      | port_label('output',4,'armDone');
      | port_label('output',5,'armFault');
      | port_label('output',6,'vacuum');
      | port_label('output',7,'c1');
      | port_label('output',8,'c2');
      | port_label('output',9,'c3');
      | port_label('output',10,'r1');
      | port_label('output',11,'r2');
      | port_label('output',12,'r3');
      | port_label('output',13,'d1');
      | port_label('output',14,'d2');
      | port_label('output',15,'d3');
      | port_label('output',16,'percValid');
      | port_label('output',17,'moreBoxes');
      | port_label('output',18,'scanDone');
      | port_label('output',19,'finish');
      | port_label('output',20,'needHome');
  Need Home Delay : UnitDelay  InitialCondition=false  SampleTime=0.02  HasFrameUpgradeWarning=on
  Perception Valid Delay : UnitDelay  InitialCondition=false  SampleTime=0.02  HasFrameUpgradeWarning=on
  Pose To Robot Transform : MATLAB Function  TreatAsAtomicUnit=on
  Robot Kinova : robotsim3dlib/Simulation 3D Robot  Priority=2  actorInputType=RigidBodyTree Object  RigidBodyTree=gen3  ActorName=Ro2Kinova  existActorChekBox=off  initialTrans=[0 0 0]  initialRot=[0 0 0]  initialConfig=qStow  EndEffector=ToolTip  eeOffsetInpChekBox=off  eeTargetTrans=[-0.04 0 0.245]  eeTargetRot=[0 1.2217 3.1416]  enableRegionGraspChekBox=on  regionGraspInpChekBox=on  eeTargTransDiff=[0.2 0.2 0.2]  eeTargRotDiff=[0 0 0]  inpConfEnbVal=on  inpGraspEnbVal=on  inpTransEnbVal=on  outConfEnbVal=on  outGraspEnbVal=on  outTransEnbVal=off  SampleTime=0.02  ActorType=SimulinkVehicle  ID=C  aMode=6  ActorTag=Ro2Kinova  Mesh=RigidBodyTree
  Robot Out Unused 1 : Terminator
  Robot Out Unused 2 : Terminator
  Robot Pack : MATLAB Function  TreatAsAtomicUnit=on
  RobotTaskFSM : Stateflow chart  TreatAsAtomicUnit=on
  Scan Done Delay : UnitDelay  InitialCondition=false  SampleTime=0.02  HasFrameUpgradeWarning=on
  Sense Bus Delay : UnitDelay  InitialCondition=zeros(1,8)  SampleTime=0.02  HasFrameUpgradeWarning=on
  Target Actor : Constant  Value=uint8('TargetBox')  OutDataTypeStr=uint8
  Target Actor uint8 : DataTypeConversion  OutDataTypeStr=uint8  SaturateOnIntegerOverflow=off  RndMeth=Floor
  Term_Differential_Drive_Kinematics_2 : Terminator
  Term_RobotTaskFSM_7 : Terminator
  Term_RobotTaskFSM_8 : Terminator
  Velocity Split : Demux  Outputs=2
  Pose : Outport
  Pack : Outport  Port=2
  Lift : Outport  Port=3
  State : Outport  Port=4
  wires:
  Navigation Arm Controller/3 -> AtGoal Delay/1
  AtGoal Delay/1 -> RobotTaskFSM/1(AtGoal)
  Navigation Arm Controller/4 -> ArmDone Delay/1
  ArmDone Delay/1 -> RobotTaskFSM/2(ArmDone)
  Navigation Arm Controller/5 -> Arm Fault Delay/1
  Arm Fault Delay/1 -> RobotTaskFSM/8(ArmFault)
  Navigation Arm Controller/6 -> Grasped Delay/1
  Grasped Delay/1 -> RobotTaskFSM/7(IsTargetGrasped), Navigation Arm Controller/8
  Navigation Arm Controller/16 -> Perception Valid Delay/1
  Perception Valid Delay/1 -> RobotTaskFSM/3(PerceptionValid)
  Navigation Arm Controller/17 -> More Boxes Delay/1
  More Boxes Delay/1 -> RobotTaskFSM/9(MoreBoxes)
  Navigation Arm Controller/18 -> Scan Done Delay/1
  Scan Done Delay/1 -> RobotTaskFSM/10(ScanDone)
  Navigation Arm Controller/19 -> Finish Delay/1
  Finish Delay/1 -> RobotTaskFSM/11(Finish)
  Navigation Arm Controller/20 -> Need Home Delay/1
  Need Home Delay/1 -> RobotTaskFSM/12(NeedHome)
  Box Coord Zero 1/1 -> RobotTaskFSM/4(BoxX)
  Box Coord Zero 2/1 -> RobotTaskFSM/5(BoxY)
  Box Coord Zero 3/1 -> RobotTaskFSM/6(BoxZ)
  RobotTaskFSM/1(TaskState) -> Navigation Arm Controller/1, State/1
  RobotTaskFSM/2(GoalX) -> Navigation Arm Controller/2
  RobotTaskFSM/3(GoalY) -> Navigation Arm Controller/3
  RobotTaskFSM/4(IKTargetX) -> Navigation Arm Controller/4
  RobotTaskFSM/5(IKTargetY) -> Navigation Arm Controller/5
  RobotTaskFSM/6(IKTargetZ) -> Navigation Arm Controller/6
  EstPose/1 -> Navigation Arm Controller/7
  SenseBus/1 -> Sense Bus Delay/1
  Sense Bus Delay/1 -> Navigation Arm Controller/10
  CamBus/1 -> Cam Bus Delay/1
  Cam Bus Delay/1 -> Navigation Arm Controller/11
  Base Pose Delay/1 -> Navigation Arm Controller/12, Pose/1, Pose To Robot Transform/1(pose)
  Navigation Arm Controller/8 -> Idx Select/1(c2), Robot Pack/4(c2)
  Idx Select/1(idx) -> Idx Delay/1
  Idx Delay/1 -> Box Meas Pick/2(idx)
  Pool/1 -> Box Meas Pick/1(pool)
  Box Meas Pick/1(y) -> Navigation Arm Controller/9
  Navigation Arm Controller/7 -> Robot Pack/1(c)
  Navigation Arm Controller/10 -> Robot Pack/2(r)
  Navigation Arm Controller/13 -> Robot Pack/3(d)
  Robot Pack/1(y) -> Pack/1
  Navigation Arm Controller/2 -> Lift Select/1(q), Robot Kinova/1
  Lift Select/1(y) -> Lift/1
  Navigation Arm Controller/9 -> Ctl Unused 9/1
  Navigation Arm Controller/11 -> Ctl Unused 11/1
  Navigation Arm Controller/12 -> Ctl Unused 12/1
  Navigation Arm Controller/14 -> Ctl Unused 14/1
  Navigation Arm Controller/15 -> Ctl Unused 15/1
  Navigation Arm Controller/1 -> Velocity Split/1
  Velocity Split/1 -> Differential Drive Kinematics/1
  Velocity Split/2 -> Differential Drive Kinematics/2
  Differential Drive Kinematics/1 -> Base Pose Delay/1
  Target Actor/1 -> Target Actor uint8/1
  Pose To Robot Transform/1(translation) -> Robot Kinova/2
  Pose To Robot Transform/2(rotation) -> Robot Kinova/3
  Target Actor uint8/1 -> Robot Kinova/4
  Native Grasp Off/1 -> Robot Kinova/5
  Grasp Translation/1 -> Robot Kinova/6
  Grasp Rotation/1 -> Robot Kinova/7
  Robot Kinova/1 -> Robot Out Unused 1/1
  Robot Kinova/2 -> Robot Out Unused 2/1
  Differential Drive Kinematics/2 -> Term_Differential_Drive_Kinematics_2/1
  RobotTaskFSM/7(GraspCmd) -> Term_RobotTaskFSM_7/1
  RobotTaskFSM/8(PlaceCmd) -> Term_RobotTaskFSM_8/1
